simulink model "FCSMPC_double_vector_2025b"  (R2025b)
settings: Solver=FixedStepDiscrete  StartTime=0.0  StopTime=2  FixedStep=SimulinkTs  RelTol=1e-3
PreLoadFcn:
  | % Verzeichnis des Modells zum MATLAB-Pfad hinzufügen
  | modelDir = fileparts(get_param(bdroot, 'FileName'));
  | addpath(modelDir);
  | 
  | % Nur der Dateiname – kein Pfad!
  | set_param(bdroot, 'DataDictionary', 'FOC_params.sldd');
model workspace (MAT data in the model file):
  Np : Simulink.Parameter (value not decoded)
values from neighbouring files (symbols this model uses):
  Filter_Current_FilterTimeConst = 3.3333333333333335E-5    [FOC_params.sldd]
  Filter_Current_SensorTimeConst = 1.5915494309189535E-6    [FOC_params.sldd]
  FOC = evalin("base", "FOC")    [createFOC_SLDD.m]
  FOC_Control_Current_KIid = 10.0    [FOC_params.sldd]
  FOC_Control_Current_KIiq = 10.0    [FOC_params.sldd]
  FOC_Control_Current_KPid = 0.20418507462686566    [FOC_params.sldd]
  FOC_Control_Current_KPiq = 0.58674626865671642    [FOC_params.sldd]
  FOC_Control_Current_Krd = 0.8    [FOC_params.sldd]
  FOC_Control_Current_Krq = 0.8    [FOC_params.sldd]
  FOC_Control_Current_TclCur = 0.1    [FOC_params.sldd]
  FOC_Control_Current_Tnd = 0.1    [FOC_params.sldd]
  FOC_Control_Current_Tnq = 0.1    [FOC_params.sldd]
  FOC_Control_InverterVdc_V = 400.0    [FOC_params.sldd]
  FOC_Control_MotorImax_A = 650.0    [FOC_params.sldd]
  FOC_Control_MTPA_MTPV_nT_id_grid = -450.06704889786266 -439.56177000270145 -427.77784873303676 -416.66404703197372 -406.07553272717422 -395.15516533678584 -384.31176061747851 -374.03652088128132 -363.90551910193739 -353.79478643334204 -344.0221683092833 -334.51243453441936 -324.94614350292119 -315.21793409137081 -305.26543360965195 -295.21828280911944 -285.133916324101 -275.01232812136521 -264.86951532374729 -254.7797625148454 -244    [FOC_params.sldd]
  FOC_Control_MTPA_MTPV_nT_iq_grid = -449.09165648258488 -442.56958748923387 -437.25247759546528 -430.91792082419158 -423.83735797306491 -417.11730433547 -410.54064621830616 -403.71584331167304 -396.93611069310379 -390.15794305727007 -382.97216593027133 -375.44639668848538 -367.93447385667577 -360.57088856352266 -353.41289778449368 -346.34020584402072 -339.28416684923008 -332.22010880540631 -325.11927997033376 -317.92299905654966 -31    [FOC_params.sldd]
  FOC_Control_MTPA_MTPV_T_vec = -245.0 -240.0 -235.0 -230.0 -225.0 -220.0 -215.0 -210.0 -205.0 -200.0 -195.0 -190.0 -185.0 -180.0 -175.0 -170.0 -165.0 -160.0 -155.0 -150.0 -145.0 -140.0 -135.0 -130.0 -125.0 -120.0 -115.0 -110.0 -105.0 -100.0 -95.0 -90.0 -85.0 -80.0 -75.0 -70.0 -65.0 -60.0 -55.0 -50.0 -45.0 -40.0 -35.0 -30.0 -25.0 -20.0 -15.0 -10.0 -5.0 0.0 5.0 10.0 15.0 20.0 25.0 30.0 35.0 40.0 45.0 50.0 55.0 60.0 65.0 70.0 75.0    [FOC_params.sldd]
  FOC_Control_MTPA_MTPV_w_vec = 0.0 10.471975511965978 20.943951023931955 31.415926535897931 41.887902047863911 52.359877559829883 62.831853071795862 73.303828583761828 83.775804095727821 94.247779607693786 104.71975511965977 115.19173063162575 125.66370614359172 136.1356816555577 146.60765716752366 157.07963267948966 167.55160819145564 178.02358370342159 188.49555921538757 198.96753472735358 209.43951023931953 219.9114857512855    [FOC_params.sldd]
  FOC_Control_OpenLoop_Id_Ref_A = 0.0    [FOC_params.sldd]
  FOC_Control_OpenLoop_Iq_Ref_A = 0.0    [FOC_params.sldd]
  FOC_Control_OpenLoop_Ud_OpenLoop_V = 0.0    [FOC_params.sldd]
  FOC_Control_OpenLoop_Uq_OpenLoop_V = 0.0    [FOC_params.sldd]
  FOC_Control_RF_omegamech_rad_s = 3141.5926535897934    [FOC_params.sldd]
  FOC_Control_RF_RateCurrent_A = 500.0    [FOC_params.sldd]
  FOC_Control_RF_RateTrq_Nm = 500.0    [FOC_params.sldd]
  FOC_Control_theta_mechOffsetFix = 0.0    [FOC_params.sldd]
  FOC_Control_theta_mechOffsetTime = 0.0    [FOC_params.sldd]
  FOC_Control_TorqueRef_Nm = 10.0    [FOC_params.sldd]
  FOC_Control_Umax_V = 230.94010767585033    [FOC_params.sldd]
  FOC_Flag_ClosedLoopControl = 1.0    [FOC_params.sldd]
  FOC_Flag_ControlStrategy = 2.0    [FOC_params.sldd]
  FOC_Flag_PWMEnable = 1.0    [FOC_params.sldd]
  FOC_Flag_ResetControl = 0.0    [FOC_params.sldd]
  FOC_Flag_TorqueControl = 1.0    [FOC_params.sldd]
  FOC_LUT_DQLimiter_DQ_LUTScaling = 1.8749999999999995E-5    [FOC_params.sldd]
  FOC_PWM_AZSPWMMethod = 3.0    [FOC_params.sldd]
  FOC_PWM_HybridMode = 1.0    [FOC_params.sldd]
  FOC_PWM_LB1 = 0.5    [FOC_params.sldd]
  FOC_PWM_LB2 = 0.77    [FOC_params.sldd]
  FOC_PWM_PWMManuel = 1.0    [FOC_params.sldd]
  FOC_PWM_RSPWMMethod = 2.0    [FOC_params.sldd]
  FOC_PWM_UB1 = 0.66    [FOC_params.sldd]
  FOC_PWM_UB2 = 0.9    [FOC_params.sldd]
  FOC_SampleTime_TsCur = 0.0001    [FOC_params.sldd]
undefined symbols (not defined in the file or in its folder): dspblkCoreblockFVToolHelper, FCS, Filter, gcbh, Plant, SimulinkTs
libraries: hdlsllib x2, simulink x2, autolibfluxpmsm x1
(part 3 of 8)

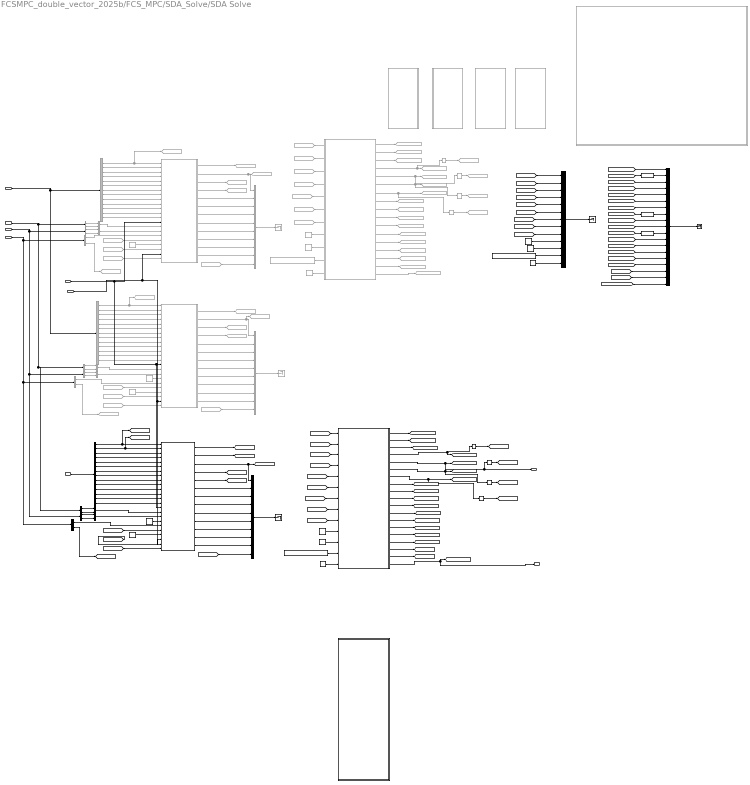
== system FCSMPC_double_vector_2025b/FCS_MPC/SDA_Solve/SDA Solve ==
  idiq_fb_A : Inport
  idiq_ref : Inport  Port=2
  ModelMatrix : Inport  Port=3
  ModelMatrix_hybrid : Inport  Port=4
  FCS_Param : Inport  Port=5
  Iabc_Motor : Inport  Port=6
  Sin_Cos_Theta_Current : Inport  Port=7
  " SDA_Solve_Synchronized" : MATLAB Function  Commented=on  TreatAsAtomicUnit=on
  " SDA_Solve_Synchronized1" : MATLAB Function  TreatAsAtomicUnit=on
  " SDA_Solve_Synchronized2" : MATLAB Function  TreatAsAtomicUnit=on
  Bus Creator1 : BusCreator  Commented=on  Inputs=10
  Bus Creator2 : BusCreator  Commented=on  Inputs=10
  Bus Creator3 : BusCreator  Inputs=13
  Bus Creator4 : BusCreator  Inputs=10
  Bus Selector : BusSelector  Commented=on  OutputSignals=idref,iqref
  Bus Selector1 : BusSelector  Commented=on  OutputSignals=Id_fb_A,Iq_fb_A
  Bus Selector10 : BusSelector  OutputSignals=H_exp,H_emb,Gamma,Phi,Lambdafsw_SE,Upsil,Bd,Bs_TI,deltaIdqBaseOffset,deltaIdqState,magnitudeGain,phaseCompensation,rippleAttenuation,rippleDelay
  Bus Selector11 : BusSelector  OutputSignals=FCS_Ts_SDA_D_V,FCS_NmaxNode
  Bus Selector2 : BusSelector  Commented=on  OutputSignals=idref,iqref
  Bus Selector3 : BusSelector  Commented=on  OutputSignals=H,Gamma,Phi,Lambdafsw_SE,Upsil,Bd,Bs_TI,deltaIdqBaseOffset,deltaIdqState,magnitudeGain,phaseCompensation,rippleAttenuation,rippleDelay
  Bus Selector4 : BusSelector  Commented=on  OutputSignals=FCS_Ts_SDA_D_V,FCS_NmaxNode
  Bus Selector5 : BusSelector  Commented=on  OutputSignals=Id_fb_A,Iq_fb_A
  Bus Selector6 : BusSelector  Commented=on  OutputSignals=H,Gamma,Phi,Lambdafsw_SE,Upsil,Bd,Bs_TI,deltaIdqBaseOffset,deltaIdqState,magnitudeGain,phaseCompensation,rippleAttenuation,rippleDelay
  Bus Selector7 : BusSelector  Commented=on  OutputSignals=FCS_Ts_SDA_D_V,FCS_NmaxNode
  Bus Selector8 : BusSelector  OutputSignals=idref,iqref
  Bus Selector9 : BusSelector  OutputSignals=Id_fb_A,Iq_fb_A
  Constant1 : Constant  Commented=on  Value=1e4
  Constant10 : Constant  Value=10
  Constant{6..8,13..14} (5 alike) : Constant  Value=1e4
  Constant15 : Constant  Value=FOC.SampleTime.BSW.DeadTime/FCS.Ts_SDA*2
  Constant16 : Constant  Value=10
  Constant2 : Constant  Commented=on  Value=1e4
  Constant3 : Constant  Commented=on  Value=1e4
  Constant4 : Constant  Commented=on  Value=FOC.SampleTime.BSW.DeadTime/FCS.Ts_SDA*2
  Constant5 : Constant  Commented=on  Value=10
  Constant9 : Constant  Value=FOC.SampleTime.BSW.DeadTime/FCS.Ts_SDA*2
  Controller_Delay : Constant  Commented=on  Value=0
  Controller_Delay1 : Constant  Commented=on  Value=0
  Controller_Delay2 : Constant  Value=0
  Delay1 : Delay  DelayLength=1  InitialCondition=zeros(15,1)
  Delay2 : Delay  Commented=on  DelayLength=1  InitialCondition=zeros(15,1)
  Delay3 : Delay  Commented=on  DelayLength=1  InitialCondition=zeros(3,1)
  Delay4 : Delay  Commented=on  DelayLength=1  InitialCondition=false
  Delay5 : Delay  Commented=on  DelayLength=1  InitialCondition=zeros(6,1)
  Delay6 : Delay  DelayLength=1  InitialCondition=zeros(3,1)
  Delay7 : Delay  DelayLength=1  InitialCondition=false
  Delay8 : Delay  DelayLength=1  InitialCondition=zeros(6,1)
  From{,7,32,35} (4 alike) : From  Commented=on  GotoTag=iabcPredictedPrevious
  From1 : From  Commented=on  GotoTag=U_applied
  From10 : From  Commented=on  GotoTag=U_unc
  From2 : From  Commented=on  GotoTag=Uopt_prev
  From3 : From  Commented=on  GotoTag=predictionValid
  From33 : From  Commented=on  GotoTag=U_applied
  From34 : From  Commented=on  GotoTag=predictionValid
  From4 : From  Commented=on  GotoTag=deltaabcBase
  From5 : From  Commented=on  GotoTag=deltaabcSwitch
  From6 : From  Commented=on  GotoTag=Nmax
  From8 : From  Commented=on  GotoTag=iabcReconstruction
  From9 : From  Commented=on  GotoTag=H
  Goto : Goto  Commented=on  GotoTag=iabcPredictedPrevious
  Goto1 : Goto  Commented=on  GotoTag=U_applied
  Goto10 : Goto  Commented=on  GotoTag=deltaabcBase
  Goto11 : Goto  Commented=on  GotoTag=deltaabcSwitch
  Goto12 : Goto  Commented=on  GotoTag=Nmax
  Goto13 : Goto  Commented=on  GotoTag=iabcReconstruction
  Goto14 : Goto  Commented=on  GotoTag=H
  Goto15 : Goto  Commented=on  GotoTag=U_unc
  Goto2 : Goto  Commented=on  GotoTag=Uopt_prev
  Goto3 : Goto  Commented=on  GotoTag=predictionValid
  Goto4 : Goto  Commented=on  GotoTag=deltaabcBase
  Goto5 : Goto  Commented=on  GotoTag=deltaabcSwitch
  Goto6 : Goto  Commented=on  GotoTag=Nmax
  Goto7 : Goto  Commented=on  GotoTag=iabcReconstruction
  Goto8 : Goto  Commented=on  GotoTag=H
  Goto9 : Goto  Commented=on  GotoTag=U_unc
  Goto_ref_Jbabai : Goto  Commented=on  GotoTag=sda_reference_Jbabai
  Goto_ref_Jopt : Goto  Commented=on  GotoTag=sda_reference_Jopt
  Goto_ref_Jround : Goto  Commented=on  GotoTag=sda_reference_Jround
  Goto_ref_Jshift : Goto  Commented=on  GotoTag=sda_reference_Jshift
  Goto_ref_Uapply : Goto  Commented=on  GotoTag=sda_reference_Uapply
  Goto_ref_Uopt : Goto  Commented=on  GotoTag=sda_reference_Uopt
  Goto_ref_bestCMVCost : Goto  Commented=on  GotoTag=sda_reference_bestCMVCost
  Goto_ref_cmvMetricRatio : Goto  Commented=on  GotoTag=sda_reference_cmvMetricRatio
  Goto_ref_debug_lower : Goto  Commented=on  GotoTag=sda_reference_debug_lower
  Goto_ref_debug_upper : Goto  Commented=on  GotoTag=sda_reference_debug_upper
  Goto_ref_iabcPredictedNext : Goto  Commented=on  GotoTag=sda_reference_iabcPredictedNext
  Goto_ref_leafNodes : Goto  Commented=on  GotoTag=sda_reference_leafNodes
  Goto_ref_nodes : Goto  Commented=on  GotoTag=sda_reference_nodes
  Goto_ref_optimal : Goto  Commented=on  GotoTag=sda_reference_optimal
  Goto_ref_predictionValidNext : Goto  Commented=on  GotoTag=sda_reference_predictionValidNext
  Goto_ref_solutionToggle : Goto  Commented=on  GotoTag=sda_reference_solutionToggle
  Goto_ref_switchCountApplied : Goto  Commented=on  GotoTag=sda_reference_switchCountApplied
  No_Compensation : MATLAB Function  Commented=on  TreatAsAtomicUnit=on
  PSPL_TestFrame : Subsystem  Commented=on
  QP_Runtime_40k_Simplified : MATLAB Function  Commented=on  TreatAsAtomicUnit=on
  QP_Runtime_40k_Simplified_Hybrid : MATLAB Function  TreatAsAtomicUnit=on
  QP_Runtime_40k_Simplified_embedded_H : MATLAB Function  Commented=on  TreatAsAtomicUnit=on
  Ref_leafNodes_uint1 : DataTypeConversion  OutDataTypeStr=uint32  SaturateOnIntegerOverflow=off  RndMeth=Floor
  Ref_nodes_uint1 : DataTypeConversion  OutDataTypeStr=uint32  SaturateOnIntegerOverflow=off  RndMeth=Floor
  Ref_switchCountApplied_uint1 : DataTypeConversion  OutDataTypeStr=uint32  SaturateOnIntegerOverflow=off  RndMeth=Floor
  Reference_Result_Bus1 : BusCreator  Inputs=19
  Reference_Result_Log1 : Terminator
  Scope1 : Terminator  Commented=on
  Scope2 : Terminator
  Scope3 : Terminator  Commented=on
  Scope4 : Terminator
  Vector Concatenate{,1..3} (4 alike) : Concatenate  Commented=on
  Vector Concatenate4 : Concatenate
  Vector Concatenate5 : Concatenate
  direct_feedthrough : MATLAB Function  Commented=on  TreatAsAtomicUnit=on
  original : MATLAB Function  Commented=on  TreatAsAtomicUnit=on
  simplified : MATLAB Function  Commented=on  TreatAsAtomicUnit=on
  Uapply : Outport
  solution Toggle : Outport  Port=2
  wires:
  Bus Selector4/2 -> Goto6/1  "<FCS_NmaxNode>"
  Constant3/1 -> " SDA_Solve_Synchronized"/9(lambdaDeadtime)
  " SDA_Solve_Synchronized"/7(iabcPredictedNext) -> Delay3/1, Goto_ref_iabcPredictedNext/1  "iabcPredictedNext"
  " SDA_Solve_Synchronized"/5(Uapply) -> Delay5/1, Goto_ref_Uapply/1  "Uapply"
  Constant5/1 -> " SDA_Solve_Synchronized"/11(currentEpsMargin)
  Constant2/1 -> " SDA_Solve_Synchronized"/8(lambdaZero)
  Delay2/1 -> Goto2/1  "Uopt_prev"
  Constant4/1 -> " SDA_Solve_Synchronized"/10(deadtime_ratio)
  " SDA_Solve_Synchronized"/6(predictionValidNext) -> Delay4/1, Goto_ref_predictionValidNext/1  "predictionValidNext"
  " SDA_Solve_Synchronized"/4(Uopt) -> Delay2/1, Goto_ref_Uopt/1  "Uopt"
  Delay5/1 -> Goto1/1  "U_applied"
  Delay3/1 -> Goto/1  "iabcPredictedPrevious"
  Delay4/1 -> Goto3/1  "predictionValid"
  Bus Creator1/1 -> Scope1/1  "Current_Reconstruction_Diagnose"
  " SDA_Solve_Synchronized"/17(solutionToggle) -> Goto_ref_solutionToggle/1  "solutionToggle"
  Bus Selector4/1 -> QP_Runtime_40k_Simplified/17(Ts)  "<FCS_Ts_SDA_D_V>"
  Controller_Delay/1 -> QP_Runtime_40k_Simplified/19(controllerDelay)
  QP_Runtime_40k_Simplified/1(U_unc) -> Goto9/1
  QP_Runtime_40k_Simplified/2(iabcReconstruction) -> Bus Creator1/1, Goto7/1
  QP_Runtime_40k_Simplified/3(deltaIabcBase) -> Goto4/1
  QP_Runtime_40k_Simplified/4(deltaIabcSwitch) -> Goto5/1
  QP_Runtime_40k_Simplified/5(predictionError) -> Bus Creator1/2
  QP_Runtime_40k_Simplified/6(reconstructionError) -> Bus Creator1/3
  QP_Runtime_40k_Simplified/7(predictionError_dq) -> Bus Creator1/4
  QP_Runtime_40k_Simplified/8(reconstructionError_dq) -> Bus Creator1/5
  QP_Runtime_40k_Simplified/9(iabcAverageEstimated) -> Bus Creator1/6
  QP_Runtime_40k_Simplified/10(iabcRippleEstimated) -> Bus Creator1/7
  QP_Runtime_40k_Simplified/11(rippleResidual) -> Bus Creator1/8
  QP_Runtime_40k_Simplified/12(iabcSwitchCorrectionRaw) -> Bus Creator1/9
  From/1 -> QP_Runtime_40k_Simplified/20(iabcPredictedPrevious)
  From1/1 -> QP_Runtime_40k_Simplified/18(U_applied)
  From2/1 -> " SDA_Solve_Synchronized"/4(UoptPrev)
  From3/1 -> QP_Runtime_40k_Simplified/22(predictionValid)
  From6/1 -> " SDA_Solve_Synchronized"/3(NmaxNod)
  From4/1 -> " SDA_Solve_Synchronized"/6(deltaIabcBase)
  From5/1 -> " SDA_Solve_Synchronized"/7(deltaIabcSwitch)
  From7/1 -> Bus Creator1/10
  Bus Selector/1 -> Vector Concatenate/1  "<idref>"
  Bus Selector/2 -> Vector Concatenate/2  "<iqref>"
  Vector Concatenate/1 -> QP_Runtime_40k_Simplified/16(idiq_ref)
  Vector Concatenate1/1 -> QP_Runtime_40k_Simplified/15(idiqFiltered)
  Bus Selector1/2 -> Vector Concatenate1/2  "<Iq_fb_A>"
  Bus Selector1/1 -> Vector Concatenate1/1  "<Id_fb_A>"
  Bus Selector3/1 -> Goto8/1, QP_Runtime_40k_Simplified/1(H)  "<H>"
  Bus Selector3/2 -> QP_Runtime_40k_Simplified/2(Gamma)  "<Gamma>"
  Bus Selector3/3 -> QP_Runtime_40k_Simplified/3(Phi)  "<Phi>"
  Bus Selector3/4 -> QP_Runtime_40k_Simplified/4(Lambdafsw_SE)  "<Lambdafsw_SE>"
  Bus Selector3/5 -> QP_Runtime_40k_Simplified/5(Upsil)  "<Upsil>"
  Bus Selector3/6 -> QP_Runtime_40k_Simplified/6(Bd)  "<Bd>"
  Bus Selector3/7 -> QP_Runtime_40k_Simplified/7(Bs_TI)  "<Bs_TI>"
  Bus Selector3/8 -> QP_Runtime_40k_Simplified/8(deltaIdqBaseOffset)  "<deltaIdqBaseOffset>"
  Bus Selector3/9 -> QP_Runtime_40k_Simplified/9(deltaIdqState)  "<deltaIdqState>"
  Bus Selector3/10 -> QP_Runtime_40k_Simplified/10(magnitudeGain)  "<magnitudeGain>"
  Bus Selector3/11 -> QP_Runtime_40k_Simplified/11(phaseCompensation)  "<phaseCompensation>"
  Bus Selector3/12 -> QP_Runtime_40k_Simplified/12(rippleAttenuation)  "<rippleAttenuation>"
  Bus Selector3/13 -> QP_Runtime_40k_Simplified/13(rippleDelay)  "<rippleDelay>"
  From9/1 -> " SDA_Solve_Synchronized"/1(H)
  From8/1 -> " SDA_Solve_Synchronized"/5(iabcCompensated)
  From10/1 -> " SDA_Solve_Synchronized"/2(U_unc)
  Constant13/1 -> Bus Creator3/10
  Constant15/1 -> Bus Creator3/12
  Constant14/1 -> Bus Creator3/11
  [Uopt_prev] -> Bus Creator3/6
  [deltaabcBase] -> Bus Creator3/8
  Constant16/1 -> Bus Creator3/13
  [deltaabcSwitch] -> Bus Creator3/9
  [Nmax] -> Bus Creator3/5
  [H_exp] -> Bus Creator3/1
  [U_unc_exp] -> Bus Creator3/2
  [iabcReconstruction] -> Bus Creator3/7
  Bus Creator3/1 -> Scope2/1  "SDA_input"
  Reference_Result_Bus1/1 -> Reference_Result_Log1/1  "SDA_reference_output"
  " SDA_Solve_Synchronized"/1(Jopt) -> Goto_ref_Jopt/1  "Jopt"
  [sda_reference_Jopt] -> Reference_Result_Bus1/1
  " SDA_Solve_Synchronized"/2(nodes) -> Goto_ref_nodes/1  "nodes"
  [sda_reference_nodes] -> Ref_nodes_uint1/1
  Ref_nodes_uint1/1 -> Reference_Result_Bus1/2  "nodes"
  " SDA_Solve_Synchronized"/3(optimal) -> Goto_ref_optimal/1  "optimal"
  [sda_reference_optimal] -> Reference_Result_Bus1/3
  [sda_reference_Uopt] -> Reference_Result_Bus1/4
  [sda_reference_Uapply] -> Reference_Result_Bus1/5
  [sda_reference_predictionValidNext] -> Reference_Result_Bus1/6
  [sda_reference_iabcPredictedNext] -> Reference_Result_Bus1/7
  " SDA_Solve_Synchronized"/8(leafNodes) -> Goto_ref_leafNodes/1  "leafNodes"
  [sda_reference_leafNodes] -> Ref_leafNodes_uint1/1
  Ref_leafNodes_uint1/1 -> Reference_Result_Bus1/8  "leafNodes"
  " SDA_Solve_Synchronized"/9(bestCMVCost) -> Goto_ref_bestCMVCost/1  "bestCMVCost"
  [sda_reference_bestCMVCost] -> Reference_Result_Bus1/9
  " SDA_Solve_Synchronized"/10(cmvMetricRatio) -> Goto_ref_cmvMetricRatio/1  "cmvMetricRatio"
  [sda_reference_cmvMetricRatio] -> Reference_Result_Bus1/10
  " SDA_Solve_Synchronized"/11(switchCountApplied) -> Goto_ref_switchCountApplied/1  "switchCountApplied"
  [sda_reference_switchCountApplied] -> Ref_switchCountApplied_uint1/1
  Ref_switchCountApplied_uint1/1 -> Reference_Result_Bus1/11  "switchCountApplied"
  " SDA_Solve_Synchronized"/12(debug_lower) -> Goto_ref_debug_lower/1  "debug_lower"
  [sda_reference_debug_lower] -> Reference_Result_Bus1/12
  " SDA_Solve_Synchronized"/13(debug_upper) -> Goto_ref_debug_upper/1  "debug_upper"
  [sda_reference_debug_upper] -> Reference_Result_Bus1/13
  " SDA_Solve_Synchronized"/14(Jround) -> Goto_ref_Jround/1  "Jround"
  [sda_reference_Jround] -> Reference_Result_Bus1/14
  " SDA_Solve_Synchronized"/15(Jshift) -> Goto_ref_Jshift/1  "Jshift"
  [sda_reference_Jshift] -> Reference_Result_Bus1/15
  [sda_reference_solutionToggle] -> Reference_Result_Bus1/19
  Bus Selector6/13 -> QP_Runtime_40k_Simplified_embedded_H/13(rippleDelay)  "<rippleDelay>"
  Bus Selector6/12 -> QP_Runtime_40k_Simplified_embedded_H/12(rippleAttenuation)  "<rippleAttenuation>"
  Bus Selector6/11 -> QP_Runtime_40k_Simplified_embedded_H/11(phaseCompensation)  "<phaseCompensation>"
  Bus Selector6/10 -> QP_Runtime_40k_Simplified_embedded_H/10(magnitudeGain)  "<magnitudeGain>"
  Bus Selector6/9 -> QP_Runtime_40k_Simplified_embedded_H/9(deltaIdqState)  "<deltaIdqState>"
  Bus Selector6/8 -> QP_Runtime_40k_Simplified_embedded_H/8(deltaIdqBaseOffset)  "<deltaIdqBaseOffset>"
  Bus Selector6/7 -> QP_Runtime_40k_Simplified_embedded_H/7(Bs_TI)  "<Bs_TI>"
  Bus Selector6/6 -> QP_Runtime_40k_Simplified_embedded_H/6(Bd)  "<Bd>"
  Bus Selector6/5 -> QP_Runtime_40k_Simplified_embedded_H/5(Upsil)  "<Upsil>"
  Bus Selector6/4 -> QP_Runtime_40k_Simplified_embedded_H/4(Lambdafsw_SE)  "<Lambdafsw_SE>"
  Bus Selector6/3 -> QP_Runtime_40k_Simplified_embedded_H/3(Phi)  "<Phi>"
  Bus Selector6/2 -> QP_Runtime_40k_Simplified_embedded_H/2(Gamma)  "<Gamma>"
  Bus Selector6/1 -> QP_Runtime_40k_Simplified_embedded_H/1(H), Goto14/1  "<H>"
  Bus Selector5/1 -> Vector Concatenate3/1  "<Id_fb_A>"
  Bus Selector5/2 -> Vector Concatenate3/2  "<Iq_fb_A>"
  Vector Concatenate3/1 -> QP_Runtime_40k_Simplified_embedded_H/15(idiqFiltered)
  Vector Concatenate2/1 -> QP_Runtime_40k_Simplified_embedded_H/16(idiq_ref)
  Bus Selector2/2 -> Vector Concatenate2/2  "<iqref>"
  Bus Selector2/1 -> Vector Concatenate2/1  "<idref>"
  From35/1 -> Bus Creator2/10
  From34/1 -> QP_Runtime_40k_Simplified_embedded_H/23(predictionValid)
  From33/1 -> QP_Runtime_40k_Simplified_embedded_H/19(U_applied)
  From32/1 -> QP_Runtime_40k_Simplified_embedded_H/21(iabcPredictedPrevious)
  QP_Runtime_40k_Simplified_embedded_H/12(iabcSwitchCorrectionRaw) -> Bus Creator2/9
  QP_Runtime_40k_Simplified_embedded_H/11(rippleResidual) -> Bus Creator2/8
  QP_Runtime_40k_Simplified_embedded_H/10(iabcRippleEstimated) -> Bus Creator2/7
  QP_Runtime_40k_Simplified_embedded_H/9(iabcAverageEstimated) -> Bus Creator2/6
  QP_Runtime_40k_Simplified_embedded_H/8(reconstructionError_dq) -> Bus Creator2/5
  QP_Runtime_40k_Simplified_embedded_H/7(predictionError_dq) -> Bus Creator2/4
  QP_Runtime_40k_Simplified_embedded_H/6(reconstructionError) -> Bus Creator2/3
  QP_Runtime_40k_Simplified_embedded_H/5(predictionError) -> Bus Creator2/2
  QP_Runtime_40k_Simplified_embedded_H/4(deltaIabcSwitch) -> Goto11/1
  QP_Runtime_40k_Simplified_embedded_H/3(deltaIabcBase) -> Goto10/1
  QP_Runtime_40k_Simplified_embedded_H/2(iabcReconstruction) -> Goto13/1, Bus Creator2/1
  QP_Runtime_40k_Simplified_embedded_H/1(U_unc) -> Goto15/1
  Controller_Delay1/1 -> QP_Runtime_40k_Simplified_embedded_H/20(controllerDelay)
  Bus Selector7/1 -> QP_Runtime_40k_Simplified_embedded_H/18(Ts)  "<FCS_Ts_SDA_D_V>"
  Bus Creator2/1 -> Scope3/1  "Current_Reconstruction_Diagnose"
  Bus Selector7/2 -> Goto12/1  "<FCS_NmaxNode>"
  ModelMatrix/1 -> Bus Selector6/1, Bus Selector3/1
  " SDA_Solve_Synchronized"/16(Jbabai) -> Goto_ref_Jbabai/1
  [sda_reference_Jbabai] -> Reference_Result_Bus1/16
  Constant1/1 -> QP_Runtime_40k_Simplified_embedded_H/17(lambdaZeroEmbedded)
  Constant6/1 -> QP_Runtime_40k_Simplified_Hybrid/18(lambdaZeroEmbedded)
  FCS_Param/1 -> Bus Selector11/1, Bus Selector7/1, Bus Selector4/1
  Bus Selector11/2 -> [Nmax]  "<FCS_NmaxNode>"
  Bus Creator4/1 -> Scope4/1  "Current_Reconstruction_Diagnose"
  Bus Selector11/1 -> QP_Runtime_40k_Simplified_Hybrid/19(Ts)  "<FCS_Ts_SDA_D_V>"
  Iabc_Motor/1 -> QP_Runtime_40k_Simplified/21(Iabc_Motor), QP_Runtime_40k_Simplified_Hybrid/23(Iabc_Motor), QP_Runtime_40k_Simplified_embedded_H/22(Iabc_Motor)
  Controller_Delay2/1 -> QP_Runtime_40k_Simplified_Hybrid/21(controllerDelay)
  QP_Runtime_40k_Simplified_Hybrid/1(U_unc_exp) -> [U_unc_exp]
  QP_Runtime_40k_Simplified_Hybrid/3(iabcReconstruction) -> [iabcReconstruction], Bus Creator4/1
  QP_Runtime_40k_Simplified_Hybrid/4(deltaIabcBase) -> [deltaabcBase]
  QP_Runtime_40k_Simplified_Hybrid/5(deltaIabcSwitch) -> [deltaabcSwitch]
  QP_Runtime_40k_Simplified_Hybrid/6(predictionError) -> Bus Creator4/2
  QP_Runtime_40k_Simplified_Hybrid/7(reconstructionError) -> Bus Creator4/3
  QP_Runtime_40k_Simplified_Hybrid/8(predictionError_dq) -> Bus Creator4/4
  QP_Runtime_40k_Simplified_Hybrid/9(reconstructionError_dq) -> Bus Creator4/5
  QP_Runtime_40k_Simplified_Hybrid/10(iabcAverageEstimated) -> Bus Creator4/6
  QP_Runtime_40k_Simplified_Hybrid/11(iabcRippleEstimated) -> Bus Creator4/7
  QP_Runtime_40k_Simplified_Hybrid/12(rippleResidual) -> Bus Creator4/8
  QP_Runtime_40k_Simplified_Hybrid/13(iabcSwitchCorrectionRaw) -> Bus Creator4/9
  [iabcPredictedPrevious] -> QP_Runtime_40k_Simplified_Hybrid/22(iabcPredictedPrevious)
  [U_applied] -> QP_Runtime_40k_Simplified_Hybrid/20(U_applied)
  [predictionValid] -> QP_Runtime_40k_Simplified_Hybrid/24(predictionValid)
  [iabcPredictedPrevious] -> Bus Creator4/10
  idiq_ref/1 -> Bus Selector8/1, Bus Selector2/1, Bus Selector/1
  Bus Selector8/1 -> Vector Concatenate4/1  "<idref>"
  Bus Selector8/2 -> Vector Concatenate4/2  "<iqref>"
  Vector Concatenate4/1 -> QP_Runtime_40k_Simplified_Hybrid/17(idiq_ref)
  Vector Concatenate5/1 -> QP_Runtime_40k_Simplified_Hybrid/16(idiqFiltered)
  Bus Selector9/2 -> Vector Concatenate5/2  "<Iq_fb_A>"
  Bus Selector9/1 -> Vector Concatenate5/1  "<Id_fb_A>"
  idiq_fb_A/1 -> Bus Selector9/1, Bus Selector5/1, Bus Selector1/1
  Bus Selector10/1 -> [H_exp], QP_Runtime_40k_Simplified_Hybrid/1(H_exp)  "<H_exp>"
  Bus Selector10/3 -> QP_Runtime_40k_Simplified_Hybrid/3(Gamma)  "<Gamma>"
  Bus Selector10/4 -> QP_Runtime_40k_Simplified_Hybrid/4(Phi)  "<Phi>"
  Bus Selector10/5 -> QP_Runtime_40k_Simplified_Hybrid/5(Lambdafsw_SE)  "<Lambdafsw_SE>"
  Bus Selector10/6 -> QP_Runtime_40k_Simplified_Hybrid/6(Upsil)  "<Upsil>"
  Bus Selector10/7 -> QP_Runtime_40k_Simplified_Hybrid/7(Bd)  "<Bd>"
  Bus Selector10/8 -> QP_Runtime_40k_Simplified_Hybrid/8(Bs_TI)  "<Bs_TI>"
  Bus Selector10/9 -> QP_Runtime_40k_Simplified_Hybrid/9(deltaIdqBaseOffset)  "<deltaIdqBaseOffset>"
  Bus Selector10/10 -> QP_Runtime_40k_Simplified_Hybrid/10(deltaIdqState)  "<deltaIdqState>"
  Bus Selector10/11 -> QP_Runtime_40k_Simplified_Hybrid/11(magnitudeGain)  "<magnitudeGain>"
  Bus Selector10/12 -> QP_Runtime_40k_Simplified_Hybrid/12(phaseCompensation)  "<phaseCompensation>"
  Bus Selector10/13 -> QP_Runtime_40k_Simplified_Hybrid/13(rippleAttenuation)  "<rippleAttenuation>"
  Bus Selector10/14 -> QP_Runtime_40k_Simplified_Hybrid/14(rippleDelay)  "<rippleDelay>"
  Sin_Cos_Theta_Current/1 -> QP_Runtime_40k_Simplified/14(Sin_Cos_Theta), QP_Runtime_40k_Simplified_Hybrid/15(Sin_Cos_Theta), QP_Runtime_40k_Simplified_embedded_H/14(Sin_Cos_Theta)
  ModelMatrix_hybrid/1 -> Bus Selector10/1
  " SDA_Solve_Synchronized1"/16(JbabaiEmbedded) -> [sda_reference_Jbabai]
  " SDA_Solve_Synchronized1"/15(Jshift) -> [sda_reference_Jshift]  "Jshift"
  " SDA_Solve_Synchronized1"/14(Jround) -> [sda_reference_Jround]  "Jround"
  " SDA_Solve_Synchronized1"/13(debug_upper) -> [sda_reference_debug_upper]  "debug_upper"
  " SDA_Solve_Synchronized1"/12(debug_lower) -> [sda_reference_debug_lower]  "debug_lower"
  " SDA_Solve_Synchronized1"/11(switchCountApplied) -> [sda_reference_switchCountApplied]  "switchCountApplied"
  " SDA_Solve_Synchronized1"/10(cmvMetricRatio) -> [sda_reference_cmvMetricRatio]  "cmvMetricRatio"
  " SDA_Solve_Synchronized1"/9(bestCMVCost) -> [sda_reference_bestCMVCost]  "bestCMVCost"
  " SDA_Solve_Synchronized1"/8(leafNodes) -> [sda_reference_leafNodes]  "leafNodes"
  " SDA_Solve_Synchronized1"/3(optimal) -> [sda_reference_optimal]  "optimal"
  " SDA_Solve_Synchronized1"/2(nodes) -> [sda_reference_nodes]  "nodes"
  " SDA_Solve_Synchronized1"/1(Jopt) -> [sda_reference_Jopt]  "Jopt"
  [U_unc_exp] -> " SDA_Solve_Synchronized1"/2(U_unc_exp)
  [iabcReconstruction] -> " SDA_Solve_Synchronized1"/7(iabcCompensated)
  [H_exp] -> " SDA_Solve_Synchronized1"/1(H_exp)
  [deltaabcSwitch] -> " SDA_Solve_Synchronized1"/9(deltaIabcSwitch)
  [deltaabcBase] -> " SDA_Solve_Synchronized1"/8(deltaIabcBase)
  [Nmax] -> " SDA_Solve_Synchronized1"/5(NmaxNod)
  [Uopt_prev] -> " SDA_Solve_Synchronized1"/6(UoptPrev)
  " SDA_Solve_Synchronized1"/19(solutionToggle) -> solution Toggle/1, [sda_reference_solutionToggle]  "solutionToggle"
  Delay7/1 -> [predictionValid]  "predictionValid"
  Delay6/1 -> [iabcPredictedPrevious]  "iabcPredictedPrevious"
  Delay8/1 -> [U_applied]  "U_applied"
  " SDA_Solve_Synchronized1"/4(Uopt) -> [sda_reference_Uopt], Delay1/1  "Uopt"
  " SDA_Solve_Synchronized1"/6(predictionValidNext) -> [sda_reference_predictionValidNext], Delay7/1  "predictionValidNext"
  Constant9/1 -> " SDA_Solve_Synchronized1"/12(deadtime_ratio)
  Delay1/1 -> [Uopt_prev]  "Uopt_prev"
  Constant7/1 -> " SDA_Solve_Synchronized1"/10(lambdaZero)
  Constant10/1 -> " SDA_Solve_Synchronized1"/13(currentEpsMargin)
  " SDA_Solve_Synchronized1"/5(Uapply) -> [sda_reference_Uapply], Uapply/1, Delay8/1  "Uapply"
  " SDA_Solve_Synchronized1"/7(iabcPredictedNext) -> [sda_reference_iabcPredictedNext], Delay6/1  "iabcPredictedNext"
  Constant8/1 -> " SDA_Solve_Synchronized1"/11(lambdaDeadtime)
  Bus Selector10/2 -> [H_emb], QP_Runtime_40k_Simplified_Hybrid/2(H_emb)  "<H_emb>"
  QP_Runtime_40k_Simplified_Hybrid/2(U_unc_emb) -> [U_unc_emb]
  [H_emb] -> " SDA_Solve_Synchronized1"/3(H_emb)
  [U_unc_emb] -> " SDA_Solve_Synchronized1"/4(U_unc_emb)
  [H_emb] -> Bus Creator3/3
  [U_unc_emb] -> Bus Creator3/4
  " SDA_Solve_Synchronized1"/17(JbabaiExplicit) -> [JbabaiExplicit]
  " SDA_Solve_Synchronized1"/18(initialRadius) -> [initialRadius]
  [JbabaiExplicit] -> Reference_Result_Bus1/17
  [initialRadius] -> Reference_Result_Bus1/18

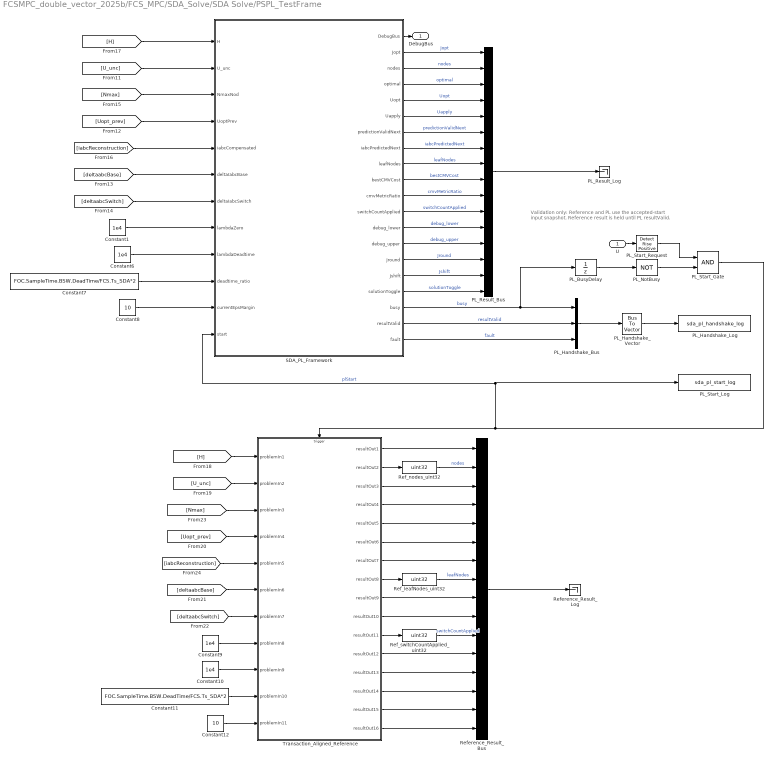
== system FCSMPC_double_vector_2025b/FCS_MPC/SDA_Solve/SDA Solve/PSPL_TestFrame ==
  note: Validation only:
      | Reference and PL use the accepted-start input snapshot.
      | Reference result is held until PL resultValid.
  U : Inport
  Constant{1,6,9..10} (4 alike) : Constant  Value=1e4
  Constant11 : Constant  Value=FOC.SampleTime.BSW.DeadTime/FCS.Ts_SDA*2
  Constant12 : Constant  Value=10
  Constant7 : Constant  Value=FOC.SampleTime.BSW.DeadTime/FCS.Ts_SDA*2
  Constant8 : Constant  Value=10
  PL_BusyDelay : UnitDelay  InitialCondition=false  SampleTime=-1  HasFrameUpgradeWarning=on
  PL_Handshake_Bus : BusCreator  Inputs=3
  PL_Handshake_Log : ToWorkspace  VariableName=sda_pl_handshake_log  SaveFormat=Structure With Time  SampleTime=-1
  PL_Handshake_Vector : BusToVector
  PL_NotBusy : Logic  Operator=NOT  AllPortsSameDT=off  OutDataTypeStr=boolean
  PL_Result_Bus : BusCreator  Inputs=16
  PL_Result_Log : Terminator
  PL_Start_Gate : Logic  AllPortsSameDT=off  OutDataTypeStr=boolean
  PL_Start_Log : ToWorkspace  VariableName=sda_pl_start_log  SaveFormat=Structure With Time  SampleTime=-1
  PL_Start_Request : simulink/Logic and Bit Operations/Detect Rise Positive  vinit=0  OutDataTypeStr=boolean
  Ref_leafNodes_uint32 : DataTypeConversion  OutDataTypeStr=uint32  SaturateOnIntegerOverflow=off  RndMeth=Floor
  Ref_nodes_uint32 : DataTypeConversion  OutDataTypeStr=uint32  SaturateOnIntegerOverflow=off  RndMeth=Floor
  Ref_switchCountApplied_uint32 : DataTypeConversion  OutDataTypeStr=uint32  SaturateOnIntegerOverflow=off  RndMeth=Floor
  Reference_Result_Bus : BusCreator  Inputs=16
  Reference_Result_Log : Terminator
  SDA_PL_Framework : Subsystem  TreatAsAtomicUnit=on
  Transaction_Aligned_Reference : Subsystem  TreatAsAtomicUnit=on
  DebugBus : Outport
  wires:
  Transaction_Aligned_Reference/1(resultOut1) -> Reference_Result_Bus/1
  Transaction_Aligned_Reference/9(resultOut9) -> Reference_Result_Bus/9
  PL_NotBusy/1 -> PL_Start_Gate/2
  [iabcReconstruction] -> SDA_PL_Framework/5(iabcCompensated)
  [U_unc] -> Transaction_Aligned_Reference/2(problemIn2)
  SDA_PL_Framework/5(Uopt) -> PL_Result_Bus/4  "Uopt"
  Transaction_Aligned_Reference/8(resultOut8) -> Ref_leafNodes_uint32/1
  Constant1/1 -> SDA_PL_Framework/8(lambdaZero)
  [H] -> SDA_PL_Framework/1(H)
  SDA_PL_Framework/17(solutionToggle) -> PL_Result_Bus/16  "solutionToggle"
  Transaction_Aligned_Reference/10(resultOut10) -> Reference_Result_Bus/10
  Constant10/1 -> Transaction_Aligned_Reference/9(problemIn9)
  SDA_PL_Framework/6(Uapply) -> PL_Result_Bus/5  "Uapply"
  Transaction_Aligned_Reference/12(resultOut12) -> Reference_Result_Bus/12
  PL_Handshake_Bus/1 -> PL_Handshake_Vector/1
  PL_Start_Request/1 -> PL_Start_Gate/1
  SDA_PL_Framework/7(predictionValidNext) -> PL_Result_Bus/6  "predictionValidNext"
  PL_Start_Gate/1 -> SDA_PL_Framework/12(start), PL_Start_Log/1, Transaction_Aligned_Reference/Trigger  "plStart"
  SDA_PL_Framework/19(resultValid) -> PL_Handshake_Bus/2  "resultValid"
  [Nmax] -> SDA_PL_Framework/3(NmaxNod)
  SDA_PL_Framework/3(nodes) -> PL_Result_Bus/2  "nodes"
  Transaction_Aligned_Reference/11(resultOut11) -> Ref_switchCountApplied_uint32/1
  SDA_PL_Framework/8(iabcPredictedNext) -> PL_Result_Bus/7  "iabcPredictedNext"
  [H] -> Transaction_Aligned_Reference/1(problemIn1)
  [deltaabcBase] -> SDA_PL_Framework/6(deltaIabcBase)
  Transaction_Aligned_Reference/15(resultOut15) -> Reference_Result_Bus/15
  Transaction_Aligned_Reference/5(resultOut5) -> Reference_Result_Bus/5
  Ref_switchCountApplied_uint32/1 -> Reference_Result_Bus/11  "switchCountApplied"
  SDA_PL_Framework/1(DebugBus) -> DebugBus/1
  [deltaabcBase] -> Transaction_Aligned_Reference/6(problemIn6)
  PL_Handshake_Vector/1 -> PL_Handshake_Log/1
  SDA_PL_Framework/10(bestCMVCost) -> PL_Result_Bus/9  "bestCMVCost"
  Constant12/1 -> Transaction_Aligned_Reference/11(problemIn11)
  Ref_leafNodes_uint32/1 -> Reference_Result_Bus/8  "leafNodes"
  Transaction_Aligned_Reference/7(resultOut7) -> Reference_Result_Bus/7
  Transaction_Aligned_Reference/3(resultOut3) -> Reference_Result_Bus/3
  SDA_PL_Framework/18(busy) -> PL_Handshake_Bus/1, PL_BusyDelay/1  "busy"
  [Uopt_prev] -> Transaction_Aligned_Reference/4(problemIn4)
  SDA_PL_Framework/12(switchCountApplied) -> PL_Result_Bus/11  "switchCountApplied"
  SDA_PL_Framework/16(Jshift) -> PL_Result_Bus/15  "Jshift"
  SDA_PL_Framework/2(Jopt) -> PL_Result_Bus/1  "Jopt"
  PL_BusyDelay/1 -> PL_NotBusy/1
  Transaction_Aligned_Reference/4(resultOut4) -> Reference_Result_Bus/4
  SDA_PL_Framework/14(debug_upper) -> PL_Result_Bus/13  "debug_upper"
  Constant8/1 -> SDA_PL_Framework/11(currentEpsMargin)
  Constant11/1 -> Transaction_Aligned_Reference/10(problemIn10)
  SDA_PL_Framework/4(optimal) -> PL_Result_Bus/3  "optimal"
  Transaction_Aligned_Reference/16(resultOut16) -> Reference_Result_Bus/16
  [Uopt_prev] -> SDA_PL_Framework/4(UoptPrev)
  [Nmax] -> Transaction_Aligned_Reference/3(problemIn3)
  [U_unc] -> SDA_PL_Framework/2(U_unc)
  Constant7/1 -> SDA_PL_Framework/10(deadtime_ratio)
  Constant9/1 -> Transaction_Aligned_Reference/8(problemIn8)
  Transaction_Aligned_Reference/13(resultOut13) -> Reference_Result_Bus/13
  SDA_PL_Framework/13(debug_lower) -> PL_Result_Bus/12  "debug_lower"
  Reference_Result_Bus/1 -> Reference_Result_Log/1
  [deltaabcSwitch] -> Transaction_Aligned_Reference/7(problemIn7)
  Transaction_Aligned_Reference/6(resultOut6) -> Reference_Result_Bus/6
  SDA_PL_Framework/20(fault) -> PL_Handshake_Bus/3  "fault"
  Transaction_Aligned_Reference/2(resultOut2) -> Ref_nodes_uint32/1
  [iabcReconstruction] -> Transaction_Aligned_Reference/5(problemIn5)
  Transaction_Aligned_Reference/14(resultOut14) -> Reference_Result_Bus/14
  Constant6/1 -> SDA_PL_Framework/9(lambdaDeadtime)
  Ref_nodes_uint32/1 -> Reference_Result_Bus/2  "nodes"
  SDA_PL_Framework/11(cmvMetricRatio) -> PL_Result_Bus/10  "cmvMetricRatio"
  PL_Result_Bus/1 -> PL_Result_Log/1
  SDA_PL_Framework/15(Jround) -> PL_Result_Bus/14  "Jround"
  SDA_PL_Framework/9(leafNodes) -> PL_Result_Bus/8  "leafNodes"
  [deltaabcSwitch] -> SDA_PL_Framework/7(deltaIabcSwitch)
  U/1 -> PL_Start_Request/1
